simulink model "2026A_A#U9898_60Hz"  (R2023b)
settings: Solver=VariableStepAuto  StartTime=0.0  StopTime=0.5  RelTol=1e-3
libraries: spsSeriesRLCBranchLib x13, spsVoltageMeasurementLib x5, spsCurrentMeasurementLib x4, spsUniversalBridgeLib x3, spsMeanLib x2, simulink x2, spsRMSLib x2, spsTHDLib x2, spsACVoltageSourceLib x1, slpidlib x1, powerlib_extras x1, spspowerguiLib x1
settings Model: SimulationMode=accelerator  Creator=abc6820292  LastModifiedBy=Codex
settings DataIOCC: ReturnWorkspaceOutputs=off
settings DebuggingCC: UnconnectedInputMsg=warning  UnconnectedOutputMsg=warning  UnconnectedLineMsg=warning
settings ModelReferenceCC: EnableRefExpFcnMdlSchedulingChecks=on
settings RTWCC: DLArmComputeVersion=19.05

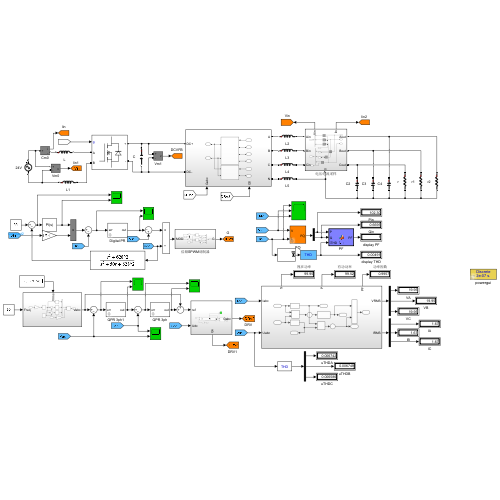
[thumbnail: Simulink's stored preview of the top-level diagram]
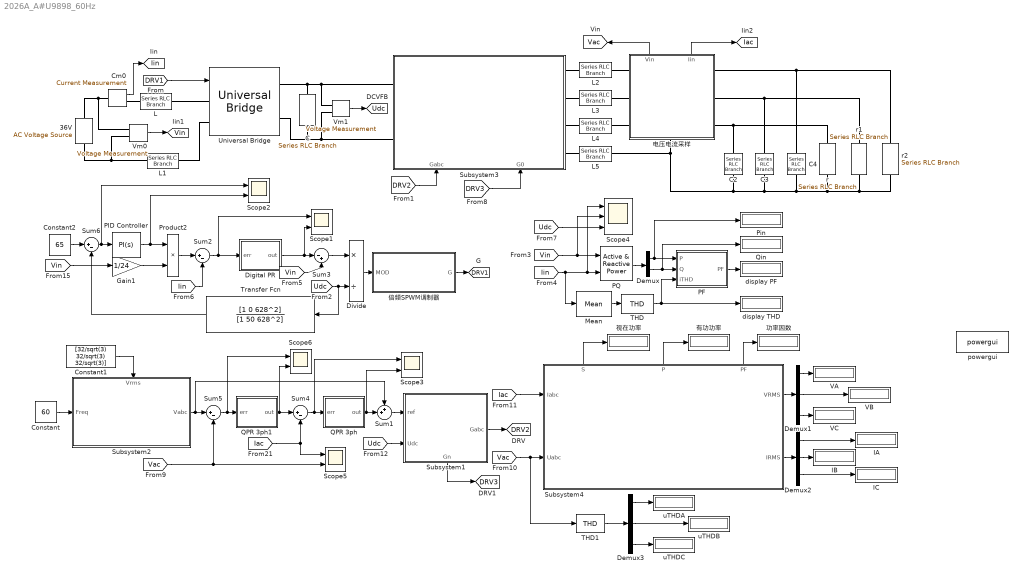
== system 2026A_A#U9898_60Hz ==
  36V : spsACVoltageSourceLib/AC Voltage Source  Amplitude=36*sqrt(2)  Phase=0  Frequency=50  SampleTime=0  Measurements=None  BusType=swing  Pref=10e3  Qref=0  Qmin=-inf  Qmax=+inf
  C : spsSeriesRLCBranchLib/Series RLC Branch  LConnTagsString=__new0  RConnTagsString=__new0  BranchType=C  Resistance=0.01  Inductance=7e-4  SetiL0=off  InitialCurrent=0  Capacitance=4e-3  Setx0=on  InitialVoltage=45  Measurements=None
  C2 : spsSeriesRLCBranchLib/Series RLC Branch  LConnTagsString=__new0  RConnTagsString=__new0  BranchType=C  Resistance=0  Inductance=0  SetiL0=off  InitialCurrent=0  Capacitance=1e-5  Setx0=off  InitialVoltage=310  Measurements=None
  C3 : spsSeriesRLCBranchLib/Series RLC Branch  LConnTagsString=__new0  RConnTagsString=__new0  BranchType=C  Resistance=0  Inductance=0  SetiL0=off  InitialCurrent=0  Capacitance=1e-5  Setx0=off  InitialVoltage=310  Measurements=None
  C4 : spsSeriesRLCBranchLib/Series RLC Branch  LConnTagsString=__new0  RConnTagsString=__new0  BranchType=C  Resistance=0  Inductance=0  SetiL0=off  InitialCurrent=0  Capacitance=1e-5  Setx0=off  InitialVoltage=310  Measurements=None
  Cm0 : spsCurrentMeasurementLib/Current Measurement  PhasorSimulation=off  OutputType=Complex  PSBequivalent=0
  Constant : Constant  Value=60
  Constant1 : Constant  Value=[32/sqrt(3) 32/sqrt(3) 32/sqrt(3)]
  Constant2 : Constant  Value=65
  Demux : Demux  Outputs=2
  Demux1 : Demux  Outputs=3
  Demux2 : Demux  Outputs=3
  Demux3 : Demux  Outputs=3
  Digital PR : Subsystem  mask{Kp=5, Kr=20, Wc=5, Ts=1/20000, Upper=400, Lower=-400}
      mask DialogControl ParameterGroupVar Prompt: 参数
  Divide : Product  Inputs=*/
  Gain1 : Gain  Gain=1/24
  IA : Display
      settings: Format=bank
  IB : Display
      settings: Format=bank
  IC : Display
      settings: Format=bank
  L : spsSeriesRLCBranchLib/Series RLC Branch  LConnTagsString=__new0  RConnTagsString=__new0  BranchType=L  Resistance=0.05  Inductance=3e-4  SetiL0=off  InitialCurrent=0  Capacitance=1e-3  Setx0=off  InitialVoltage=0  Measurements=None
  L1 : spsSeriesRLCBranchLib/Series RLC Branch  LConnTagsString=__new0  RConnTagsString=__new0  BranchType=L  Resistance=0.05  Inductance=3e-4  SetiL0=off  InitialCurrent=0  Capacitance=1e-3  Setx0=off  InitialVoltage=0  Measurements=None
  L{2..5} (4 alike) : spsSeriesRLCBranchLib/Series RLC Branch  LConnTagsString=__new0  RConnTagsString=__new0  BranchType=L  Resistance=0.05  Inductance=5e-4  SetiL0=off  InitialCurrent=0  Capacitance=1e-3  Setx0=off  InitialVoltage=0  Measurements=None
  Mean : spsMeanLib/Mean  Freq=20000  Vinit=0  Ts=0
  PF : MATLAB Function  TreatAsAtomicUnit=on
  PID Controller : slpidlib/PID Controller  Controller=PI  Form=Parallel  TimeDomain=Continuous-time  UseExternalTs=off  SampleTime=-1  IntegratorMethod=Forward Euler  FilterMethod=Forward Euler  ControllerParametersSource=internal  P=0.4  I=20  UseKiTs=off  D=0.005  N=100  UseFilter=on  TunerSelectOption=Transfer Function Based (PID Tuner App)  InitialConditionSource=internal  InitialConditionForIntegrator=0  InitialConditionForFilter=0  DifferentiatorICPrevScaledInput=0  ExternalReset=none  TrackingMode=off  Kt=1  LimitOutput=off  SatLimitsSource=internal  UpperSaturationLimit=200  LowerSaturationLimit=0  LinearizeAsGain=on  AntiWindupMode=clamping  Kb=1  LimitIntegrator=off  UpperIntegratorSaturationLimit=inf  LowerIntegratorSaturationLimit=-inf  POutMin=[]  POutMax=[]  IOutMin=[]  IOutMax=[]  DOutMin=[]  DOutMax=[]  NOutMin=[]  NOutMax=[]  SumOutMin=[]  SumOutMax=[]  SaturationOutMin=[]  SaturationOutMax=[]  PParamMin=[]  PParamMax=[]  IParamMin=[]  IParamMax=[]  DParamMin=[]  DParamMax=[]  NParamMin=[]  NParamMax=[]  KbParamMin=[]  KbParamMax=[]  KtParamMin=[]  KtParamMax=[]  KbOutMin=[]  KbOutMax=[]  KtOutMin=[]  KtOutMax=[]  IntegratorOutMin=[]  IntegratorOutMax=[]  FilterOutMin=[]  FilterOutMax=[]  SumI1OutMin=[]  SumI1OutMax=[]  SumI2OutMin=[]  SumI2OutMax=[]  SumI3OutMin=[]  SumI3OutMax=[]  SumI4OutMin=[]  SumI4OutMax=[]  SumDOutMin=[]  SumDOutMax=[]  DifferentiatorOutMin=[]  DifferentiatorOutMax=[]  FilterDiffOutCoefMin=[]  FilterDiffOutCoefMax=[]  ReciprocalOutMin=[]  ReciprocalOutMax=[]  SumDenOutMin=[]  SumDenOutMax=[]  SumNumOutMin=[]  SumNumOutMax=[]  DivideOutMin=[]  DivideOutMax=[]  UdiffTsProdOutMin=[]  UdiffTsProdOutMax=[]  NTsProdOutMin=[]  NTsProdOutMax=[]  UintegralTsProdOutMin=[]  UintegralTsProdOutMax=[]  UngainTsProdOutMin=[]  UngainTsProdOutMax=[]  ClampingZeroOutDataTypeStr=Inherit: Inherit via back propagation  ClampingZeroOutMin=[]  ClampingZeroOutMax=[]  FilterDenConstantOutDataTypeStr=Inherit: Inherit via back propagation  FilterDenConstantOutMin=[]  FilterDenConstantOutMax=[]  PCopyOutDataTypeStr=Inherit: Inherit via back propagation  PCopyOutMin=[]  PCopyOutMax=[]  NCopyOutDataTypeStr=Inherit: Inherit via back propagation  NCopyOutMin=[]  NCopyOutMax=[]  IntegratorContinuousStateAttributes=''  IntegratorStateMustResolveToSignalObject=off  IntegratorRTWStateStorageClass=Auto  FilterContinuousStateAttributes=''  FilterStateMustResolveToSignalObject=off  FilterRTWStateStorageClass=Auto  ParallelPVariant=InternalParameters  IdealPVariant=Disabled  IVariant=InternalParameters  DVariant=Disabled  IntegratorVariant=Continuous  SatVariant=Disabled  AWVariant=Passthrough  PCopyVariant=Disabled  TRVariant=Disabled  FdbkBlocksVariant=Forward  IdealPFdbkVariant=Disabled  SatFdbkVariant=Disabled  DerivativeFilterVariant=Disabled  NVariant=Disabled  NCopyVariant=Disabled_SignalSpec  FilterICVariant=Disabled  IntegratorICVariant=InternalICs  ExternalResetVariant=Disabled  TRSumVariant=Passthrough  SumFdbkVariant=Disabled  SumVariant=Sum_PI  TsampFilterVariant=InternalTs  TsampNgainVariant=Passthrough  TsampIntegralVariant=Disabled_SignalSpec  ExternalSaturationOutDataTypeStr=Inherit: Same as second input
  PQ : powerlib_extras/Measurements/Active & Reactive Power  f1=50
  Pin : Display
      settings: Format=bank
  Product2 : Product  RndMeth=Zero
  QPR 3ph : Subsystem  mask{Kp=5, Kr=50, Wc=5, Ts=1/20000, Upper=60, Lower=-60}
      mask DialogControl ParameterGroupVar Prompt: 参数
  QPR 3ph1 : Subsystem  mask{Kp=0.1, Kr=100, Wc=1, Ts=1/20000, Upper=60, Lower=-60}
      mask DialogControl ParameterGroupVar Prompt: 参数
  Qin : Display
  Scope{1..3,5..6} (5 alike) : Scope  NumInputPorts=2
  Scope4 : Scope  NumInputPorts=3
  Subsystem1 : Subsystem
      settings: PortSchema="{\"entries\":[{\"content\":{\"sides\":[{\"content\":{\"connectorIds\":[\"In1\",\"In2\"]},\"type\":\"ConnectorPlacement.EquallySpacedRectSide\",\"uuid\":\"ffbfa849-ae7e-484b-8f62-2a401a1da371\"},{\"content\":{\"connectorIds\":[\"Out1\"],\"side\":\"RIGHT\"},\"type\":\"ConnectorPlacement.EquallySpacedRectSide\",\"uuid\":\"e08180f0-b598-4732-8bbc-503d0e150e22\"},{\"content\":{\"side\":\"TOP\"},\"type\":\"ConnectorPlacement.EquallySpacedRectSide\",\"uuid\":\"4409d359-fc49-4067-ac49-474d913d3159\"},{\"content\":{\"connectorIds\":[\"Out2\"],\"side\":\"BOTTOM\"},\"type\":\"ConnectorPlacement.EquallySpacedRectSide\",\"uuid\":\"5d435d63-d38f-48d8-82d2-98313854c09c\"}]},\"type\":\"ConnectorPlacement.EquallySpacedConnector\",\"uuid\":\"7e2e8f5b-ae64-493d-8481-bf05f705a7ac\"}],\"packageUris\":[\"http://schema.mathworks.com/mf0/Connector/R2020b\"],\"version\":\"1.0\"}"
  Subsystem2 : Subsystem
      settings: PortSchema="{\"entries\":[{\"content\":{\"sides\":[{\"content\":{\"connectorIds\":[\"In1\"]},\"type\":\"ConnectorPlacement.EquallySpacedRectSide\",\"uuid\":\"b83f0250-9c61-4256-afad-581095ab140f\"},{\"content\":{\"connectorIds\":[\"Out1\"],\"side\":\"RIGHT\"},\"type\":\"ConnectorPlacement.EquallySpacedRectSide\",\"uuid\":\"e21d95d9-bd65-4b8b-8e7b-d6ad7b8ad5cc\"},{\"content\":{\"connectorIds\":[\"In2\"],\"side\":\"TOP\"},\"type\":\"ConnectorPlacement.EquallySpacedRectSide\",\"uuid\":\"3e84556d-e7a5-4296-98ac-10e766fe76c2\"}]},\"type\":\"ConnectorPlacement.EquallySpacedConnector\",\"uuid\":\"d357bca2-f059-42e0-868e-69ff40dc2149\"}],\"packageUris\":[\"http://schema.mathworks.com/mf0/Connector/R2020b\"],\"version\":\"1.0\"}"
  Subsystem3 : Subsystem
      settings: PortSchema="{\"entries\":[{\"content\":{\"sides\":[{\"content\":{\"connectorIds\":[\"LConn1\",\"LConn2\"]},\"type\":\"ConnectorPlacement.EquallySpacedRectSide\",\"uuid\":\"78b2e702-d06c-4e88-88fa-76d063fe9b62\"},{\"content\":{\"connectorIds\":[\"RConn1\",\"RConn2\",\"RConn3\",\"RConn4\"],\"side\":\"RIGHT\"},\"type\":\"ConnectorPlacement.EquallySpacedRectSide\",\"uuid\":\"7bc0c85a-fd6f-4f5e-acb5-d7baabe65af7\"},{\"content\":{\"side\":\"TOP\"},\"type\":\"ConnectorPlacement.EquallySpacedRectSide\",\"uuid\":\"08102ab6-f4c4-4a42-9468-f733ccd64290\"},{\"content\":{\"connectorIds\":[\"In1\",\"In2\"],\"side\":\"BOTTOM\"},\"type\":\"ConnectorPlacement.EquallySpacedRectSide\",\"uuid\":\"d24dfa10-9dd8-43ca-ac07-c82c5936d107\"}]},\"type\":\"ConnectorPlacement.EquallySpacedConnector\",\"uuid\":\"9f42a9a1-5471-4f27-a0ba-eb296522cfc6\"}],\"packageUris\":[\"http://schema.mathworks.com/mf0/Connector/R2020b\"],\"version\":\"1.0\"}"
  Subsystem4 : Subsystem
      settings: PortSchema="{\"entries\":[{\"content\":{\"sides\":[{\"content\":{\"connectorIds\":[\"In1\",\"In2\"]},\"type\":\"ConnectorPlacement.EquallySpacedRectSide\",\"uuid\":\"8f3b7bf1-7c44-4492-a357-aa6e3e6d66a4\"},{\"content\":{\"connectorIds\":[\"Out1\",\"Out2\"],\"side\":\"RIGHT\"},\"type\":\"ConnectorPlacement.EquallySpacedRectSide\",\"uuid\":\"7ae784cf-6bcf-4684-9c07-1770fc60c8a0\"},{\"content\":{\"connectorIds\":[\"Out3\",\"Out4\",\"Out5\"],\"side\":\"TOP\"},\"type\":\"ConnectorPlacement.EquallySpacedRectSide\",\"uuid\":\"0e016931-6232-4ad6-afe9-572a0571336f\"},{\"content\":{\"side\":\"BOTTOM\"},\"type\":\"ConnectorPlacement.EquallySpacedRectSide\",\"uuid\":\"ef67c6ee-ba81-4705-af34-81581e7e9907\"}]},\"type\":\"ConnectorPlacement.EquallySpacedConnector\",\"uuid\":\"922af512-c0ff-443f-816c-194775a78dc8\"}],\"packageUris\":[\"http://schema.mathworks.com/mf0/Connector/R2020b\"],\"version\":\"1.0\"}"
  Sum1 : Sum  Inputs=++|
  Sum{2,4..6} (4 alike) : Sum  Inputs=|+-
  Sum3 : Sum  Inputs=|-+
  THD : spsTHDLib/THD  Freq=50  Ts=0
  THD1 : spsTHDLib/THD  Freq=60  Ts=0
  Transfer Fcn : TransferFcn  Numerator=[1 0 628^2]  Denominator=[1 50 628^2]
  Universal Bridge : spsUniversalBridgeLib/Universal Bridge  Arms=2  SnubberResistance=1e5  SnubberCapacitance=1e-9  Device=MOSFET / Diodes  Ron=1e-2  Lon=0  ForwardVoltages="[  1  1  ]"  ForwardVoltage=0  GTOparameters=[ 10e-6 , 20e-6 ]  IGBTparameters=[ 1e-6 , 2e-6 ]  Measurements=None  Measurements_2=None  converterType=Rectifier
  VA : Display
      settings: Format=bank
  VB : Display
      settings: Format=bank
  VC : Display
      settings: Format=bank
  Vm0 : spsVoltageMeasurementLib/Voltage Measurement  PhasorSimulation=off  OutputType=Complex  PSBequivalent=0
  Vm1 : spsVoltageMeasurementLib/Voltage Measurement  PhasorSimulation=off  OutputType=Complex  PSBequivalent=0
  display PF : Display
  display THD : Display
  powergui : spspowerguiLib/powergui  SimulationMode=Discrete  SampleTime=2e-7  frequency=60  Iterations=50  frequencyindice=0  Pbase=100e6  ErrMax=1e-4  UnitsV=kV  UnitsW=MW  buscounter=0  FunctionMessages=off  echomessages=off  EnableUseOfTLC=off  CurrentSourceSwitches=off  DisableSnubberDevices=off  DisableRonSwitches=off  DisableVfSwitches=off  DisplayEquations=off  AutomaticDiscreteSolvers=off  SolverType=Tustin/Backward Euler (TBE)  Interpol=off  ExternalGateDelay=off  methode=off  Ts=0  x0status=blocks  SPID=off  SwTol=0  HookPort=off  NonlinearTolerance=1e-4  nMaxIteration=100  ContinueOnMaxIteration=off  RestoreLinks=warning  ResistiveCurrentMeasurement=off  Frange=[0:2:500]  Ylog=off  Xlog=on  ShowGrid=off  save=off  variable=ZData  structure=QQQQQ  ZoomFFT=off  StartTime=0.5  cycles=15  DisplayStyle=1  fundamental=60  FreqAxis=off  MaxFrequency=1000  frequencyindicesteady=1  RmsSteady=1  display=off
  r : spsSeriesRLCBranchLib/Series RLC Branch  LConnTagsString=__new0  RConnTagsString=__new0  BranchType=R  Resistance=32/(2*sqrt(3))  Inductance=12e-4  SetiL0=off  InitialCurrent=0  Capacitance=inf  Setx0=off  InitialVoltage=0  Measurements=None
  r1 : spsSeriesRLCBranchLib/Series RLC Branch  LConnTagsString=__new0  RConnTagsString=__new0  BranchType=R  Resistance=32/(2*sqrt(3))  Inductance=12e-4  SetiL0=off  InitialCurrent=0  Capacitance=inf  Setx0=off  InitialVoltage=0  Measurements=None
  r2 : spsSeriesRLCBranchLib/Series RLC Branch  LConnTagsString=__new0  RConnTagsString=__new0  BranchType=R  Resistance=32/(2*sqrt(3))  Inductance=12e-4  SetiL0=off  InitialCurrent=0  Capacitance=inf  Setx0=off  InitialVoltage=0  Measurements=None
  uTHDA : Display
  uTHDB : Display
  uTHDC : Display
  倍频SPWM调制器 : Subsystem
  功率因数 : Display
  有功功率 : Display
      settings: Format=bank
  电压电流采样 : Subsystem
      settings: PortSchema="{\"entries\":[{\"content\":{\"sides\":[{\"content\":{\"connectorIds\":[\"LConn1\",\"LConn2\",\"LConn3\"]},\"type\":\"ConnectorPlacement.EquallySpacedRectSide\",\"uuid\":\"d60dd16a-7a74-435a-96f5-79c0993f3801\"},{\"content\":{\"connectorIds\":[\"RConn1\",\"RConn2\",\"RConn3\"],\"side\":\"RIGHT\"},\"type\":\"ConnectorPlacement.EquallySpacedRectSide\",\"uuid\":\"38a0d536-50a5-43bd-9d58-6b0db9c378a0\"},{\"content\":{\"connectorIds\":[\"Out1\",\"Out2\"],\"side\":\"TOP\"},\"type\":\"ConnectorPlacement.EquallySpacedRectSide\",\"uuid\":\"65be575f-dbb8-4f94-beb1-b426df65c1d5\"},{\"content\":{\"connectorIds\":[\"RConn4\"],\"side\":\"BOTTOM\"},\"type\":\"ConnectorPlacement.EquallySpacedRectSide\",\"uuid\":\"a28dffe8-15db-4523-b673-2414d0fbe1e1\"}]},\"type\":\"ConnectorPlacement.EquallySpacedConnector\",\"uuid\":\"1fc3ca7a-50b1-4fd5-a5d3-d39cc1e6f07d\"}],\"packageUris\":[\"http://schema.mathworks.com/mf0/Connector/R2020b\"],\"version\":\"1.0\"}"
  视在功率 : Display
      settings: Format=bank
  tag scope: DRV1=global, DRV2=global, DRV3=global, Iac=global, Iin=global, Udc=global, Vac=global, Vin=global
  wires:
  Demux/1 -> Pin/1, PF/1(P)
  PF/1(PF) -> display PF/1
  Demux/2 -> Qin/1, PF/2(Q)
  PQ/1 -> Demux/1
  THD/1 -> display THD/1, PF/3(iTHD)
  [Vin] -> Scope4/2, PQ/1
  [Iin] -> Mean/1, Scope4/1, PQ/2
  Sum6/1 -> Scope2/1, PID Controller/1
  [Vin] -> Gain1/1
  [DRV1] -> Universal Bridge/1
  Vm0/1 -> [Vin]
  Cm0/1 -> [Iin]
  Vm1/1 -> [Udc]
  Constant2/1 -> Sum6/1
  Sum2/1 -> Digital PR/1(err), Scope1/1
  [Vin] -> Sum3/2
  [Udc] -> Transfer Fcn/1, Divide/2
  Digital PR/1(out) -> Scope1/2, Sum3/1
  Sum3/1 -> Divide/1
  倍频SPWM调制器/1(G) -> [DRV1]
  Divide/1 -> 倍频SPWM调制器/1(MOD)
  [Udc] -> Scope4/3
  Mean/1 -> THD/1
  PID Controller/1 -> Scope2/2, Product2/1
  Transfer Fcn/1 -> Sum6/2
  [Iin] -> Sum2/2
  Product2/1 -> Sum2/1
  Gain1/1 -> Product2/2
  [DRV2] -> Subsystem3/1(Gabc)
  [DRV3] -> Subsystem3/2(G0)
  QPR 3ph/1(out) -> Scope3/2, Sum1/2
  Sum4/1 -> Scope3/1, QPR 3ph/1(err)
  [Vac] -> Sum5/2, Scope5/2
  Subsystem2/1(Vabc) -> Sum1/1, Sum5/1
  Constant/1 -> Subsystem2/1(Freq)
  Subsystem1/2(Gn) -> [DRV3]
  Demux1/1 -> VA/1
  Subsystem4/2(IRMS) -> Demux2/1
  Sum1/1 -> Subsystem1/1(ref)
  Sum5/1 -> Scope6/1, QPR 3ph1/1(err)
  Subsystem1/1(Gabc) -> [DRV2]
  Demux1/3 -> VC/1
  [Iac] -> Sum4/2, Scope5/1
  QPR 3ph1/1(out) -> Scope6/2, Sum4/1
  Demux3/3 -> uTHDC/1
  Demux1/2 -> VB/1
  Demux2/3 -> IC/1
  [Vac] -> THD1/1, Subsystem4/2(Uabc)
  Demux3/2 -> uTHDB/1
  Subsystem4/1(VRMS) -> Demux1/1
  Demux2/1 -> IA/1
  Subsystem4/4(P) -> 有功功率/1
  Demux2/2 -> IB/1
  [Iac] -> Subsystem4/1(Iabc)
  Subsystem4/3(S) -> 视在功率/1
  Subsystem4/5(PF) -> 功率因数/1
  THD1/1 -> Demux3/1
  [Udc] -> Subsystem1/2(Udc)
  Demux3/1 -> uTHDA/1
  Constant1/1 -> Subsystem2/2(Vrms)
  电压电流采样/1(Vin) -> [Vac]
  电压电流采样/2(Iin) -> [Iac]
  connections:
  Vm0/LConn1 -- 36V/RConn1 -- Cm0/LConn1
  Vm1/LConn1 -- C/LConn1 -- Universal Bridge/RConn1 -- Subsystem3/LConn1
  Vm1/LConn2 -- Subsystem3/LConn2 -- Universal Bridge/RConn2 -- C/RConn1
  Cm0/RConn1 -- L/LConn1
  L/RConn1 -- Universal Bridge/LConn1
  Vm0/LConn2 -- 36V/LConn1 -- L1/LConn1
  L1/RConn1 -- Universal Bridge/LConn2
  L3/RConn1 -- 电压电流采样/LConn2
  L4/RConn1 -- 电压电流采样/LConn3
  L2/RConn1 -- 电压电流采样/LConn1
  Subsystem3/RConn2 -- L3/LConn1
  Subsystem3/RConn3 -- L4/LConn1
  Subsystem3/RConn1 -- L2/LConn1
  L5/LConn1 -- Subsystem3/RConn4
  L5/RConn1 -- r1/RConn1 -- r2/RConn1 -- r/RConn1 -- C4/RConn1 -- C3/RConn1 -- C2/RConn1 -- 电压电流采样/RConn4
  C2/LConn1 -- 电压电流采样/RConn3 -- r/LConn1
  C3/LConn1 -- 电压电流采样/RConn2 -- r1/LConn1
  C4/LConn1 -- 电压电流采样/RConn1 -- r2/LConn1

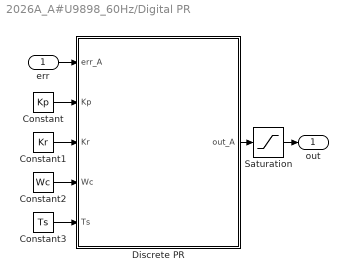
== system 2026A_A#U9898_60Hz/Digital PR ==
  err : Inport
  Constant : Constant  Value=Kp
  Constant1 : Constant  Value=Kr
  Constant2 : Constant  Value=Wc
  Constant3 : Constant  Value=Ts
  Discrete PR : MATLAB Function  TreatAsAtomicUnit=on
  Saturation : Saturate  UpperLimit=Upper  LowerLimit=Lower
  out : Outport
  wires:
  Constant1/1 -> Discrete PR/3(Kr)
  Constant3/1 -> Discrete PR/5(Ts)
  Constant/1 -> Discrete PR/2(Kp)
  Constant2/1 -> Discrete PR/4(Wc)
  Discrete PR/1(out_A) -> Saturation/1
  Saturation/1 -> out/1
  err/1 -> Discrete PR/1(err_A)

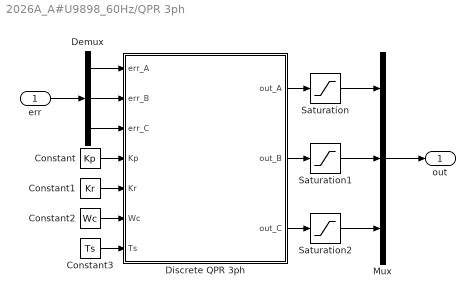
== system 2026A_A#U9898_60Hz/QPR 3ph ==
  err : Inport
  Constant : Constant  Value=Kp
  Constant1 : Constant  Value=Kr
  Constant2 : Constant  Value=Wc
  Constant3 : Constant  Value=Ts
  Demux : Demux  Outputs=3
  Discrete QPR 3ph : MATLAB Function  TreatAsAtomicUnit=on
  Mux : Mux  Inputs=3
  Saturation : Saturate  UpperLimit=Upper  LowerLimit=Lower
  Saturation1 : Saturate  UpperLimit=Upper  LowerLimit=Lower
  Saturation2 : Saturate  UpperLimit=Upper  LowerLimit=Lower
  out : Outport
  wires:
  Discrete QPR 3ph/1(out_A) -> Saturation/1
  Constant1/1 -> Discrete QPR 3ph/5(Kr)
  Constant3/1 -> Discrete QPR 3ph/7(Ts)
  Constant/1 -> Discrete QPR 3ph/4(Kp)
  Constant2/1 -> Discrete QPR 3ph/6(Wc)
  Discrete QPR 3ph/2(out_B) -> Saturation1/1
  Discrete QPR 3ph/3(out_C) -> Saturation2/1
  Demux/2 -> Discrete QPR 3ph/2(err_B)
  Demux/3 -> Discrete QPR 3ph/3(err_C)
  Demux/1 -> Discrete QPR 3ph/1(err_A)
  err/1 -> Demux/1
  Saturation2/1 -> Mux/3
  Saturation1/1 -> Mux/2
  Saturation/1 -> Mux/1
  Mux/1 -> out/1

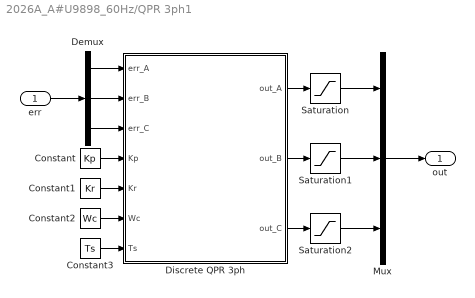
== system 2026A_A#U9898_60Hz/QPR 3ph1 ==
  err : Inport
  Constant : Constant  Value=Kp
  Constant1 : Constant  Value=Kr
  Constant2 : Constant  Value=Wc
  Constant3 : Constant  Value=Ts
  Demux : Demux  Outputs=3
  Discrete QPR 3ph : MATLAB Function  TreatAsAtomicUnit=on
  Mux : Mux  Inputs=3
  Saturation : Saturate  UpperLimit=Upper  LowerLimit=Lower
  Saturation1 : Saturate  UpperLimit=Upper  LowerLimit=Lower
  Saturation2 : Saturate  UpperLimit=Upper  LowerLimit=Lower
  out : Outport
  wires:
  Mux/1 -> out/1
  Saturation/1 -> Mux/1
  Saturation1/1 -> Mux/2
  Saturation2/1 -> Mux/3
  err/1 -> Demux/1
  Demux/1 -> Discrete QPR 3ph/1(err_A)
  Demux/3 -> Discrete QPR 3ph/3(err_C)
  Demux/2 -> Discrete QPR 3ph/2(err_B)
  Discrete QPR 3ph/3(out_C) -> Saturation2/1
  Discrete QPR 3ph/2(out_B) -> Saturation1/1
  Constant2/1 -> Discrete QPR 3ph/6(Wc)
  Constant/1 -> Discrete QPR 3ph/4(Kp)
  Constant3/1 -> Discrete QPR 3ph/7(Ts)
  Constant1/1 -> Discrete QPR 3ph/5(Kr)
  Discrete QPR 3ph/1(out_A) -> Saturation/1

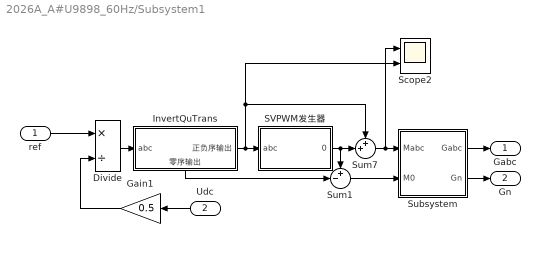
== system 2026A_A#U9898_60Hz/Subsystem1 ==
  ref : Inport
  Udc : Inport  Port=2
  Divide : Product  Inputs=*/
  Gain1 : Gain  Gain=0.5
  InvertQuTrans : Subsystem
      settings: PortSchema="{\"entries\":[{\"content\":{\"sides\":[{\"content\":{\"connectorIds\":[\"In1\"]},\"type\":\"ConnectorPlacement.EquallySpacedRectSide\",\"uuid\":\"3b0106b0-bc54-45a9-b05d-3eecf0326883\"},{\"content\":{\"connectorIds\":[\"Out1\"],\"side\":\"RIGHT\"},\"type\":\"ConnectorPlacement.EquallySpacedRectSide\",\"uuid\":\"76c8a7af-655d-43f9-845b-6e9ed12f5cd0\"},{\"content\":{\"side\":\"TOP\"},\"type\":\"ConnectorPlacement.EquallySpacedRectSide\",\"uuid\":\"5a7dd780-9a84-4f31-b60b-773284e010b3\"},{\"content\":{\"connectorIds\":[\"Out2\"],\"side\":\"BOTTOM\"},\"type\":\"ConnectorPlacement.EquallySpacedRectSide\",\"uuid\":\"2999e992-75c6-4257-aa5c-d5eb578ed629\"}]},\"type\":\"ConnectorPlacement.EquallySpacedConnector\",\"uuid\":\"db37e23d-1e3d-4a27-a575-89b3ce02feb9\"}],\"packageUris\":[\"http://schema.mathworks.com/mf0/Connector/R2020b\"],\"version\":\"1.0\"}"
  SVPWM发生器 : Subsystem
  Scope2 : Scope  NumInputPorts=2
  Subsystem : Subsystem
  Sum1 : Sum  Inputs=+-|
  Sum7 : Sum  Inputs=++|
  Gabc : Outport
  Gn : Outport  Port=2
  wires:
  ref/1 -> Divide/1
  Subsystem/1(Gabc) -> Gabc/1
  Sum7/1 -> Scope2/1, Subsystem/1(Mabc)
  InvertQuTrans/2(零序输出) -> Sum1/2
  Divide/1 -> InvertQuTrans/1(abc)
  InvertQuTrans/1(正负序输出) -> SVPWM发生器/1(abc), Scope2/2, Sum7/1
  Subsystem/2(Gn) -> Gn/1
  Sum1/1 -> Subsystem/2(M0)
  Udc/1 -> Gain1/1
  Gain1/1 -> Divide/2
  SVPWM发生器/1(0) -> Sum1/1, Sum7/2

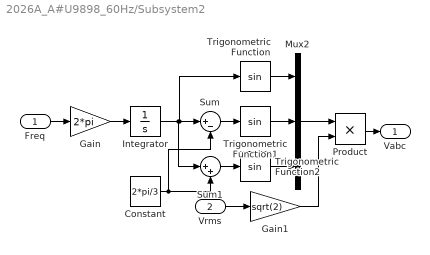
== system 2026A_A#U9898_60Hz/Subsystem2 ==
  Freq : Inport
  Vrms : Inport  Port=2
  Constant : Constant  Value=2*pi/3
  Gain : Gain  Gain=2*pi
  Gain1 : Gain  Gain=sqrt(2)
  Integrator : Integrator  WrapState=on  WrappedStateUpperValue=2*pi  WrappedStateLowerValue=0
  Mux2 : Mux  Inputs=3
  Product : Product
  Sum : Sum  Inputs=|+-
  Sum1 : Sum  Inputs=|++
  Trigonometric Function : Trigonometry
  Trigonometric Function1 : Trigonometry
  Trigonometric Function2 : Trigonometry
  Vabc : Outport
  wires:
  Gain/1 -> Integrator/1
  Freq/1 -> Gain/1
  Integrator/1 -> Sum1/1, Trigonometric Function/1, Sum/1
  Constant/1 -> Sum1/2, Sum/2
  Sum/1 -> Trigonometric Function1/1
  Sum1/1 -> Trigonometric Function2/1
  Vrms/1 -> Gain1/1
  Trigonometric Function/1 -> Mux2/1
  Trigonometric Function1/1 -> Mux2/2
  Trigonometric Function2/1 -> Mux2/3
  Mux2/1 -> Product/1
  Gain1/1 -> Product/2
  Product/1 -> Vabc/1

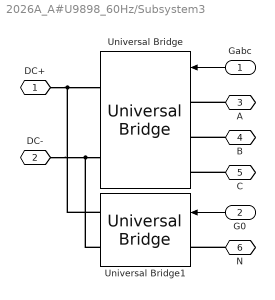
== system 2026A_A#U9898_60Hz/Subsystem3 ==
  Gabc : Inport
  G0 : Inport  Port=2
  Universal Bridge : spsUniversalBridgeLib/Universal Bridge  Arms=3  SnubberResistance=1e5  SnubberCapacitance=inf  Device=MOSFET / Diodes  Ron=1e-3  Lon=0  ForwardVoltages="[  0  0  ]"  ForwardVoltage=0  GTOparameters=[ 10e-6 , 20e-6 ]  IGBTparameters=[ 1e-6 , 2e-6 ]  Measurements=None  Measurements_2=None  converterType=Rectifier
  Universal Bridge1 : spsUniversalBridgeLib/Universal Bridge  Arms=1  SnubberResistance=1e5  SnubberCapacitance=inf  Device=MOSFET / Diodes  Ron=1e-3  Lon=0  ForwardVoltages="[  0  0  ]"  ForwardVoltage=0  GTOparameters=[ 10e-6 , 20e-6 ]  IGBTparameters=[ 1e-6 , 2e-6 ]  Measurements=None  Measurements_2=None  converterType=Rectifier
  DC+ : PMIOPort  Side=Left
  DC- : PMIOPort  Port=2  Side=Left
  A : PMIOPort  Port=3  Side=Right
  B : PMIOPort  Port=4  Side=Right
  C : PMIOPort  Port=5  Side=Right
  N : PMIOPort  Port=6  Side=Right
  wires:
  Gabc/1 -> Universal Bridge/1
  G0/1 -> Universal Bridge1/1
  connections:
  B/RConn1 -- Universal Bridge/LConn2
  C/RConn1 -- Universal Bridge/LConn3
  DC+/RConn1 -- Universal Bridge/RConn1 -- Universal Bridge1/RConn1
  DC-/RConn1 -- Universal Bridge1/RConn2 -- Universal Bridge/RConn2
  A/RConn1 -- Universal Bridge/LConn1
  N/RConn1 -- Universal Bridge1/LConn1

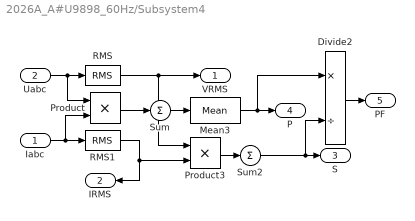
== system 2026A_A#U9898_60Hz/Subsystem4 ==
  Iabc : Inport
  Uabc : Inport  Port=2
  Divide2 : Product  Inputs=*/
  Mean3 : spsMeanLib/Mean  Freq=50  Vinit=0  Ts=0
  Product : Product
  Product3 : Product
  RMS : spsRMSLib/RMS  TrueRMS=on  Freq=50  RMSInit=0  Ts=0
  RMS1 : spsRMSLib/RMS  TrueRMS=on  Freq=50  RMSInit=0  Ts=0
  Sum : Sum  Inputs=+
  Sum2 : Sum  Inputs=+
  VRMS : Outport
  IRMS : Outport  Port=2
  S : Outport  Port=3
  P : Outport  Port=4
  PF : Outport  Port=5
  wires:
  Iabc/1 -> Product/2, RMS1/1
  RMS/1 -> VRMS/1, Product3/1
  RMS1/1 -> Product3/2, IRMS/1
  Divide2/1 -> PF/1
  Mean3/1 -> Divide2/1, P/1
  Sum/1 -> Mean3/1
  Uabc/1 -> RMS/1, Product/1
  Product/1 -> Sum/1
  Product3/1 -> Sum2/1
  Sum2/1 -> Divide2/2, S/1

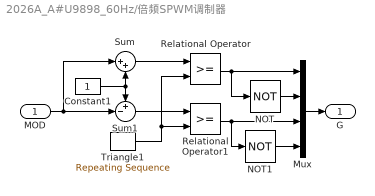
== system 2026A_A#U9898_60Hz/倍频SPWM调制器 ==
  MOD : Inport
  Constant1 : Constant
  Mux : Mux
  NOT : Logic  Operator=NOT  IconShape=distinctive  AllPortsSameDT=off  OutDataTypeStr=boolean
  NOT1 : Logic  Operator=NOT  IconShape=distinctive  AllPortsSameDT=off  OutDataTypeStr=boolean
  Relational Operator : RelationalOperator  OutDataTypeStr=boolean  InputSameDT=off
  Relational Operator1 : RelationalOperator  OutDataTypeStr=boolean  InputSameDT=off
  Sum : Sum  Inputs=|++
  Sum1 : Sum  Inputs=+-|
  Triangle1 : simulink/Sources/Repeating Sequence  rep_seq_t=[0 1/10000/2 1/10000]  rep_seq_y=[0 2 0]
  G : Outport
  wires:
  NOT1/1 -> Mux/4
  Relational Operator1/1 -> NOT1/1, Mux/3
  MOD/1 -> Sum1/2, Sum/1
  NOT/1 -> Mux/2
  Relational Operator/1 -> NOT/1, Mux/1
  Mux/1 -> G/1
  Triangle1/1 -> Relational Operator/2, Relational Operator1/2
  Sum/1 -> Relational Operator/1
  Sum1/1 -> Relational Operator1/1
  Constant1/1 -> Sum1/1, Sum/2

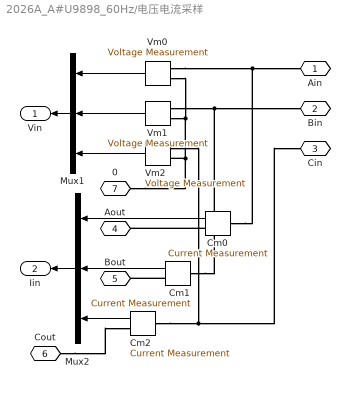
== system 2026A_A#U9898_60Hz/电压电流采样 ==
  Cm0 : spsCurrentMeasurementLib/Current Measurement  PhasorSimulation=off  OutputType=Complex  PSBequivalent=0
  Cm1 : spsCurrentMeasurementLib/Current Measurement  PhasorSimulation=off  OutputType=Complex  PSBequivalent=0
  Cm2 : spsCurrentMeasurementLib/Current Measurement  PhasorSimulation=off  OutputType=Complex  PSBequivalent=0
  Mux1 : Mux  Inputs=3
  Mux2 : Mux  Inputs=3
  Vm0 : spsVoltageMeasurementLib/Voltage Measurement  PhasorSimulation=off  OutputType=Complex  PSBequivalent=0
  Vm1 : spsVoltageMeasurementLib/Voltage Measurement  PhasorSimulation=off  OutputType=Complex  PSBequivalent=0
  Vm2 : spsVoltageMeasurementLib/Voltage Measurement  PhasorSimulation=off  OutputType=Complex  PSBequivalent=0
  Ain : PMIOPort  Side=Left
  Bin : PMIOPort  Port=2  Side=Left
  Cin : PMIOPort  Port=3  Side=Left
  Aout : PMIOPort  Port=4  Side=Right
  Bout : PMIOPort  Port=5  Side=Right
  Cout : PMIOPort  Port=6  Side=Right
  0 : PMIOPort  Port=7  Side=Right
  Vin : Outport
  Iin : Outport  Port=2
  wires:
  Cm2/1 -> Mux2/3
  Vm1/1 -> Mux1/2
  Cm1/1 -> Mux2/2
  Vm2/1 -> Mux1/3
  Vm0/1 -> Mux1/1
  Mux1/1 -> Vin/1
  Cm0/1 -> Mux2/1
  Mux2/1 -> Iin/1
  connections:
  Vm1/LConn1 -- Cm1/LConn1 -- Bin/RConn1
  Cm0/RConn1 -- Aout/RConn1
  Vm0/LConn1 -- Cm0/LConn1 -- Ain/RConn1
  Cm2/LConn1 -- Vm2/LConn1 -- Cin/RConn1
  Cm1/RConn1 -- Bout/RConn1
  Cout/RConn1 -- Cm2/RConn1
  0/RConn1 -- Vm0/LConn2 -- Vm1/LConn2 -- Vm2/LConn2

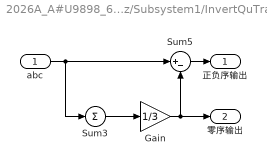
== system 2026A_A#U9898_60Hz/Subsystem1/InvertQuTrans ==
  abc : Inport
  Gain : Gain  Gain=1/3
  Sum3 : Sum  Inputs=+
  Sum5 : Sum  Inputs=|+-
  正负序输出 : Outport
  零序输出 : Outport  Port=2
  wires:
  abc/1 -> Sum5/1, Sum3/1
  Sum3/1 -> Gain/1
  Gain/1 -> Sum5/2, 零序输出/1
  Sum5/1 -> 正负序输出/1

== system 2026A_A#U9898_60Hz/Subsystem1/SVPWM发生器 ==
  abc : Inport
  Gain5 : Gain  Gain=-1/2
  MinMax : MinMax
  MinMax2 : MinMax  Function=max
  Sum1 : Sum  Inputs=|++
  0 : Outport
  wires:
  abc/1 -> MinMax/1, MinMax2/1
  MinMax/1 -> Sum1/1
  MinMax2/1 -> Sum1/2
  Sum1/1 -> Gain5/1
  Gain5/1 -> 0/1

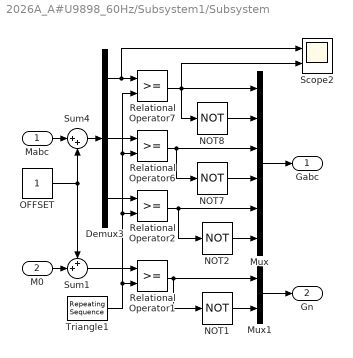
== system 2026A_A#U9898_60Hz/Subsystem1/Subsystem ==
  Mabc : Inport
  M0 : Inport  Port=2
  Demux3 : Demux  Outputs=3
  Mux : Mux  Inputs=6
  Mux1 : Mux  Inputs=2
  NOT{1..2,7..8} (4 alike) : Logic  Operator=NOT  IconShape=distinctive  AllPortsSameDT=off  OutDataTypeStr=boolean
  OFFSET : Constant
  Relational Operator{1..2,6..7} (4 alike) : RelationalOperator  OutDataTypeStr=boolean  InputSameDT=off
  Scope2 : Scope  NumInputPorts=2
  Sum1 : Sum  Inputs=++|
  Sum4 : Sum  Inputs=|++
  Triangle1 : simulink/Sources/Repeating Sequence  rep_seq_t=[0 1/20000/2 1/20000]  rep_seq_y=[0 2 0]
  Gabc : Outport
  Gn : Outport  Port=2
  wires:
  Triangle1/1 -> Relational Operator1/2, Relational Operator7/2, Relational Operator6/2, Relational Operator2/2
  Relational Operator7/1 -> NOT8/1, Scope2/2, Mux/1
  Relational Operator2/1 -> NOT2/1, Mux/5
  Relational Operator6/1 -> Mux/3, NOT7/1
  NOT8/1 -> Mux/2
  NOT7/1 -> Mux/4
  Mux/1 -> Gabc/1
  NOT2/1 -> Mux/6
  Mabc/1 -> Sum4/1
  OFFSET/1 -> Sum1/1, Sum4/2
  Sum4/1 -> Demux3/1
  Demux3/1 -> Scope2/1, Relational Operator7/1
  Demux3/2 -> Relational Operator6/1
  Demux3/3 -> Relational Operator2/1
  Mux1/1 -> Gn/1
  Relational Operator1/1 -> NOT1/1, Mux1/1
  NOT1/1 -> Mux1/2
  Sum1/1 -> Relational Operator1/1
  M0/1 -> Sum1/2

== matlab function 2026A_A#U9898_60Hz/QPR 3ph/Discrete QPR 3ph ==
  settings: updateMethod=DISCRETE  sampleTime=Ts
  data: err_A input; err_B input; err_C input; out_A output; Kp input; Kr input; Wc input; Ts input; out_B output; out_C output
function [out_A, out_B, out_C] = fcn(err_A, err_B, err_C, Kp, Kr, Wc, Ts)

W0 = 60*2*pi;

%%定义三相静态变量
persistent err_A1;
persistent err_A2;
persistent out_A1;
persistent out_A2;

persistent err_B1;
persistent err_B2;
persistent out_B1;
persistent out_B2;

persistent err_C1;
persistent err_C2;
persistent out_C1;
persistent out_C2;

%%对三相静态变量初始化
if isempty(err_A1)
    err_A1 = 0;
end
if isempty(err_A2)
    err_A2 = 0;
end
if isempty(out_A1)
    out_A1 = 0;
end
if isempty(out_A2)
    out_A2 = 0;
end

if isempty(err_B1)
    err_B1 = 0;
end
if isempty(err_B2)
    err_B2 = 0;
end
if isempty(out_B1)
    out_B1 = 0;
end
if isempty(out_B2)
    out_B2 = 0;
end

if isempty(err_C1)
    err_C1 = 0;
end
if isempty(err_C2)
    err_C2 = 0;
end
if isempty(out_C1)
    out_C1 = 0;
end
if isempty(out_C2)
    out_C2 = 0;
end

%%Discrete
t1 = Wc * Ts;
t2 = W0^2 * Ts^2;
t3 = t2 + 4*t1 + 4;

b0 = (Kp*t2 + 4*(Kp+Kr)*t1 + 4*Kp) / t3;
b1 = (2*Kp*t2 - 8*Kp) / t3;
b2 = (Kp*t2 + 4*Kp - 4*(Kp+Kr)*t1) / t3;
a1 = (2*t2 - 8) / t3;
a2 = (t2 - 4*t1 + 4) / t3;

%%计算三相输出量
out_A = b0*err_A + b1*err_A1 + b2*err_A2 - a1*out_A1 - a2*out_A2;
out_A2 = out_A1;
out_A1 = out_A;
err_A2 = err_A1;
err_A1 = err_A;

out_B = b0*err_B + b1*err_B1 + b2*err_B2 - a1*out_B1 - a2*out_B2;
out_B2 = out_B1;
out_B1 = out_B;
err_B2 = err_B1;
err_B1 = err_B;

out_C = b0*err_C + b1*err_C1 + b2*err_C2 - a1*out_C1 - a2*out_C2;
out_C2 = out_C1;
out_C1 = out_C;
err_C2 = err_C1;
err_C1 = err_C;

== matlab function 2026A_A#U9898_60Hz/PF ==
  data: P input; PF output; Q input; iTHD input
function PF = fcn(P,Q,iTHD)
% This block supports an embeddable subset of the MATLAB language.
% See the help menu for details. 
PF=(P/sqrt(P*P+Q*Q))/(sqrt(1+iTHD*iTHD));

== matlab function 2026A_A#U9898_60Hz/Digital PR/Discrete PR ==
  settings: updateMethod=DISCRETE  sampleTime=Ts
  data: err_A input; out_A output; Kp input; Kr input; Wc input; Ts input
function out_A  = fcn(err_A, Kp, Kr, Wc, Ts)

W0 = 50*2*pi;


persistent err_A1;
persistent err_A2;
persistent out_A1;
persistent out_A2;


%%对三相静态变量初始化
if isempty(err_A1)
    err_A1 = 0;
end
if isempty(err_A2)
    err_A2 = 0;
end
if isempty(out_A1)
    out_A1 = 0;
end
if isempty(out_A2)
    out_A2 = 0;
end


%%Discrete
t1 = Wc * Ts;
t2 = W0^2 * Ts^2;
t3 = t2 + 4*t1 + 4;

b0 = (Kp*t2 + 4*(Kp+Kr)*t1 + 4*Kp) / t3;
b1 = (2*Kp*t2 - 8*Kp) / t3;
b2 = (Kp*t2 + 4*Kp - 4*(Kp+Kr)*t1) / t3;
a1 = (2*t2 - 8) / t3;
a2 = (t2 - 4*t1 + 4) / t3;
%%限制输出
if b0>3000
    b0=0;
end
if b0<-3000
    b0=0;
end

%%计算输出量
out_A = b0*err_A + b1*err_A1 + b2*err_A2 - a1*out_A1 - a2*out_A2;
out_A2 = out_A1;
out_A1 = out_A;
err_A2 = err_A1;
err_A1 = err_A;

== matlab function 2026A_A#U9898_60Hz/QPR 3ph1/Discrete QPR 3ph ==
  settings: updateMethod=DISCRETE  sampleTime=Ts
  data: err_A input; err_B input; err_C input; out_A output; Kp input; Kr input; Wc input; Ts input; out_B output; out_C output
function [out_A, out_B, out_C] = fcn(err_A, err_B, err_C, Kp, Kr, Wc, Ts)

W0 = 60*2*pi;

%%定义三相静态变量
persistent err_A1;
persistent err_A2;
persistent out_A1;
persistent out_A2;

persistent err_B1;
persistent err_B2;
persistent out_B1;
persistent out_B2;

persistent err_C1;
persistent err_C2;
persistent out_C1;
persistent out_C2;

%%对三相静态变量初始化
if isempty(err_A1)
    err_A1 = 0;
end
if isempty(err_A2)
    err_A2 = 0;
end
if isempty(out_A1)
    out_A1 = 0;
end
if isempty(out_A2)
    out_A2 = 0;
end

if isempty(err_B1)
    err_B1 = 0;
end
if isempty(err_B2)
    err_B2 = 0;
end
if isempty(out_B1)
    out_B1 = 0;
end
if isempty(out_B2)
    out_B2 = 0;
end

if isempty(err_C1)
    err_C1 = 0;
end
if isempty(err_C2)
    err_C2 = 0;
end
if isempty(out_C1)
    out_C1 = 0;
end
if isempty(out_C2)
    out_C2 = 0;
end

%%Discrete
t1 = Wc * Ts;
t2 = W0^2 * Ts^2;
t3 = t2 + 4*t1 + 4;

b0 = (Kp*t2 + 4*(Kp+Kr)*t1 + 4*Kp) / t3;
b1 = (2*Kp*t2 - 8*Kp) / t3;
b2 = (Kp*t2 + 4*Kp - 4*(Kp+Kr)*t1) / t3;
a1 = (2*t2 - 8) / t3;
a2 = (t2 - 4*t1 + 4) / t3;

%%计算三相输出量
out_A = b0*err_A + b1*err_A1 + b2*err_A2 - a1*out_A1 - a2*out_A2;
out_A2 = out_A1;
out_A1 = out_A;
err_A2 = err_A1;
err_A1 = err_A;

out_B = b0*err_B + b1*err_B1 + b2*err_B2 - a1*out_B1 - a2*out_B2;
out_B2 = out_B1;
out_B1 = out_B;
err_B2 = err_B1;
err_B1 = err_B;

out_C = b0*err_C + b1*err_C1 + b2*err_C2 - a1*out_C1 - a2*out_C2;
out_C2 = out_C1;
out_C1 = out_C;
err_C2 = err_C1;
err_C1 = err_C;
